simulink model "AE200_Landing_Gear_Model"  (R2021b)
settings: Solver=VariableStepAuto  StartTime=0.0  StopTime=10.0  RelTol=1e-3
settings Model: Creator=amazgrace  LastModifiedBy=amazgrace

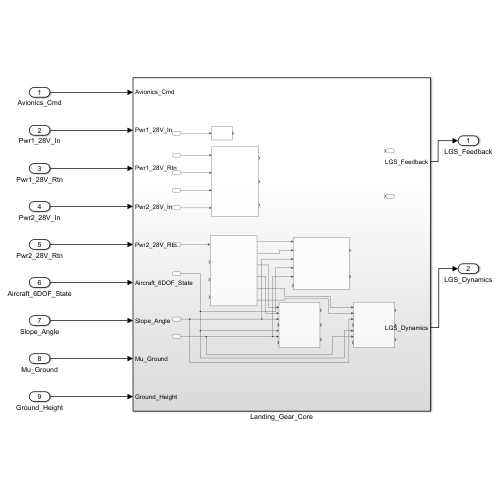
[thumbnail: Simulink's stored preview of the top-level diagram]
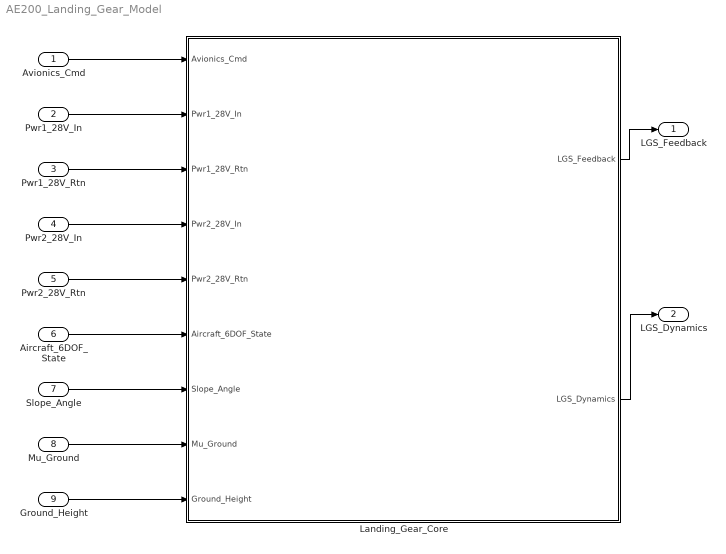
== system AE200_Landing_Gear_Model ==
  Avionics_Cmd : Inport
  Pwr1_28V_In : Inport  Port=2
  Pwr1_28V_Rtn : Inport  Port=3
  Pwr2_28V_In : Inport  Port=4
  Pwr2_28V_Rtn : Inport  Port=5
  Aircraft_6DOF_State : Inport  Port=6
  Slope_Angle : Inport  Port=7
  Mu_Ground : Inport  Port=8
  Ground_Height : Inport  Port=9
  Landing_Gear_Core : Subsystem
  LGS_Feedback : Outport
  LGS_Dynamics : Outport  Port=2
  wires:
  Avionics_Cmd/1 -> Landing_Gear_Core/1(Avionics_Cmd)
  Pwr1_28V_In/1 -> Landing_Gear_Core/2(Pwr1_28V_In)
  Pwr1_28V_Rtn/1 -> Landing_Gear_Core/3(Pwr1_28V_Rtn)
  Pwr2_28V_In/1 -> Landing_Gear_Core/4(Pwr2_28V_In)
  Pwr2_28V_Rtn/1 -> Landing_Gear_Core/5(Pwr2_28V_Rtn)
  Aircraft_6DOF_State/1 -> Landing_Gear_Core/6(Aircraft_6DOF_State)
  Landing_Gear_Core/2(LGS_Dynamics) -> LGS_Dynamics/1
  Landing_Gear_Core/1(LGS_Feedback) -> LGS_Feedback/1
  Slope_Angle/1 -> Landing_Gear_Core/7(Slope_Angle)
  Mu_Ground/1 -> Landing_Gear_Core/8(Mu_Ground)
  Ground_Height/1 -> Landing_Gear_Core/9(Ground_Height)

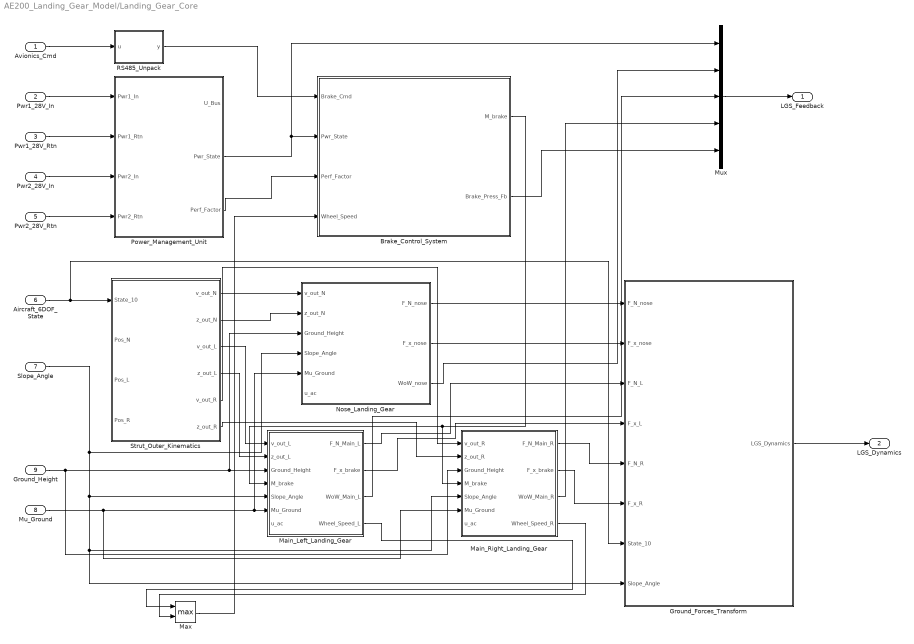
== system AE200_Landing_Gear_Model/Landing_Gear_Core ==
  Avionics_Cmd : Inport
  Pwr1_28V_In : Inport  Port=2
  Pwr1_28V_Rtn : Inport  Port=3
  Pwr2_28V_In : Inport  Port=4
  Pwr2_28V_Rtn : Inport  Port=5
  Aircraft_6DOF_State : Inport  Port=6
  Slope_Angle : Inport  Port=7
  Mu_Ground : Inport  Port=8
  Ground_Height : Inport  Port=9
  Brake_Control_System : Subsystem
  Ground_Forces_Transform : MATLAB Function  TreatAsAtomicUnit=on
  Main_Left_Landing_Gear : Subsystem
  Main_Right_Landing_Gear : Subsystem
  Max : MinMax  Function=max  Inputs=2
  Mux : Mux  Inputs=5
  Nose_Landing_Gear : Subsystem
  Power_Management_Unit : MATLAB Function  TreatAsAtomicUnit=on
  RS485_Unpack : MATLAB Function  TreatAsAtomicUnit=on
  Strut_Outer_Kinematics : MATLAB Function  TreatAsAtomicUnit=on
  LGS_Feedback : Outport
  LGS_Dynamics : Outport  Port=2
  wires:
  Avionics_Cmd/1 -> RS485_Unpack/1(u)
  Pwr1_28V_In/1 -> Power_Management_Unit/1(Pwr1_In)
  Pwr1_28V_Rtn/1 -> Power_Management_Unit/2(Pwr1_Rtn)
  Pwr2_28V_In/1 -> Power_Management_Unit/3(Pwr2_In)
  Pwr2_28V_Rtn/1 -> Power_Management_Unit/4(Pwr2_Rtn)
  Aircraft_6DOF_State/1 -> Ground_Forces_Transform/7(State_10), Strut_Outer_Kinematics/1(State_10)
  Strut_Outer_Kinematics/1(v_out_N) -> Nose_Landing_Gear/1(v_out_N)
  Strut_Outer_Kinematics/2(z_out_N) -> Nose_Landing_Gear/2(z_out_N)
  Strut_Outer_Kinematics/3(v_out_L) -> Main_Left_Landing_Gear/1(v_out_L)
  Strut_Outer_Kinematics/4(z_out_L) -> Main_Left_Landing_Gear/2(z_out_L)
  Slope_Angle/1 -> Ground_Forces_Transform/8(Slope_Angle), Main_Right_Landing_Gear/5(Slope_Angle), Main_Left_Landing_Gear/5(Slope_Angle), Nose_Landing_Gear/4(Slope_Angle)
  Strut_Outer_Kinematics/5(v_out_R) -> Main_Right_Landing_Gear/1(v_out_R)
  Strut_Outer_Kinematics/6(z_out_R) -> Main_Right_Landing_Gear/2(z_out_R)
  Mu_Ground/1 -> Nose_Landing_Gear/5(Mu_Ground), Main_Left_Landing_Gear/6(Mu_Ground), Main_Right_Landing_Gear/6(Mu_Ground)
  Ground_Height/1 -> Main_Right_Landing_Gear/3(Ground_Height), Nose_Landing_Gear/3(Ground_Height), Main_Left_Landing_Gear/3(Ground_Height)
  Nose_Landing_Gear/1(F_N_nose) -> Ground_Forces_Transform/1(F_N_nose)
  Nose_Landing_Gear/2(F_x_nose) -> Ground_Forces_Transform/2(F_x_nose)
  Main_Left_Landing_Gear/1(F_N_Main_L) -> Ground_Forces_Transform/3(F_N_L)
  Main_Left_Landing_Gear/2(F_x_brake) -> Ground_Forces_Transform/4(F_x_L)
  Main_Right_Landing_Gear/1(F_N_Main_R) -> Ground_Forces_Transform/5(F_N_R)
  Main_Right_Landing_Gear/2(F_x_brake) -> Ground_Forces_Transform/6(F_x_R)
  Ground_Forces_Transform/1(LGS_Dynamics) -> LGS_Dynamics/1
  Mux/1 -> LGS_Feedback/1
  Power_Management_Unit/2(Pwr_State) -> Brake_Control_System/2(Pwr_State), Mux/1
  Nose_Landing_Gear/3(WoW_nose) -> Mux/2
  Main_Left_Landing_Gear/3(WoW_Main_L) -> Mux/3
  Main_Right_Landing_Gear/3(WoW_Main_R) -> Mux/4
  RS485_Unpack/1(y) -> Brake_Control_System/1(Brake_Cmd)
  Power_Management_Unit/3(Perf_Factor) -> Brake_Control_System/3(Perf_Factor)
  Brake_Control_System/1(M_brake) -> Main_Right_Landing_Gear/4(M_brake), Main_Left_Landing_Gear/4(M_brake)
  Brake_Control_System/2(Brake_Press_Fb) -> Mux/5
  Main_Left_Landing_Gear/4(Wheel_Speed_L) -> Max/1
  Main_Right_Landing_Gear/4(Wheel_Speed_R) -> Max/2
  Max/1 -> Brake_Control_System/4(Wheel_Speed)

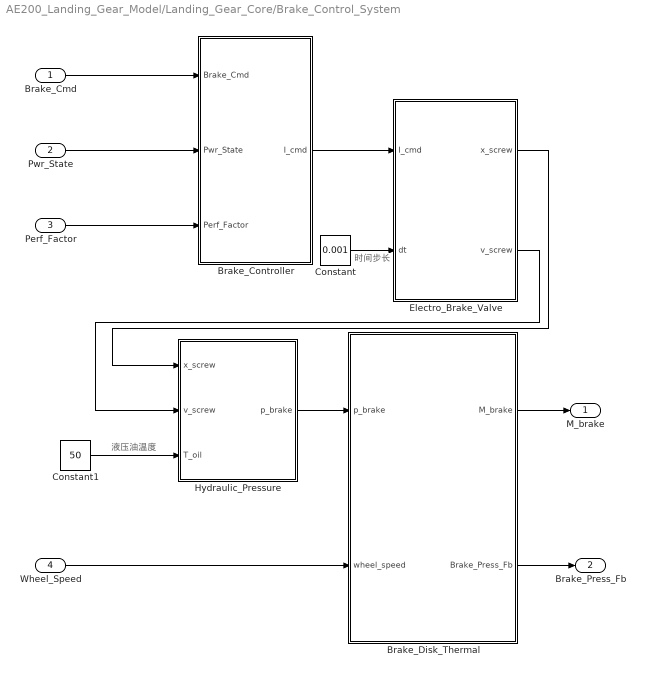
== system AE200_Landing_Gear_Model/Landing_Gear_Core/Brake_Control_System ==
  note: 时间步长
  note: 液压油温度
  Brake_Cmd : Inport
  Pwr_State : Inport  Port=2
  Perf_Factor : Inport  Port=3
  Wheel_Speed : Inport  Port=4
  Brake_Controller : MATLAB Function  TreatAsAtomicUnit=on
  Brake_Disk_Thermal : MATLAB Function  TreatAsAtomicUnit=on
  Constant : Constant  Value=0.001
  Constant1 : Constant  Value=50
  Electro_Brake_Valve : MATLAB Function  TreatAsAtomicUnit=on
  Hydraulic_Pressure : MATLAB Function  TreatAsAtomicUnit=on
  M_brake : Outport
  Brake_Press_Fb : Outport  Port=2
  wires:
  Brake_Cmd/1 -> Brake_Controller/1(Brake_Cmd)
  Pwr_State/1 -> Brake_Controller/2(Pwr_State)
  Perf_Factor/1 -> Brake_Controller/3(Perf_Factor)
  Brake_Controller/1(I_cmd) -> Electro_Brake_Valve/1(I_cmd)
  Brake_Disk_Thermal/2(Brake_Press_Fb) -> Brake_Press_Fb/1
  Brake_Disk_Thermal/1(M_brake) -> M_brake/1
  Electro_Brake_Valve/2(v_screw) -> Hydraulic_Pressure/2(v_screw)
  Hydraulic_Pressure/1(p_brake) -> Brake_Disk_Thermal/1(p_brake)
  Constant/1 -> Electro_Brake_Valve/2(dt)
  Constant1/1 -> Hydraulic_Pressure/3(T_oil)
  Wheel_Speed/1 -> Brake_Disk_Thermal/2(wheel_speed)
  Electro_Brake_Valve/1(x_screw) -> Hydraulic_Pressure/1(x_screw)

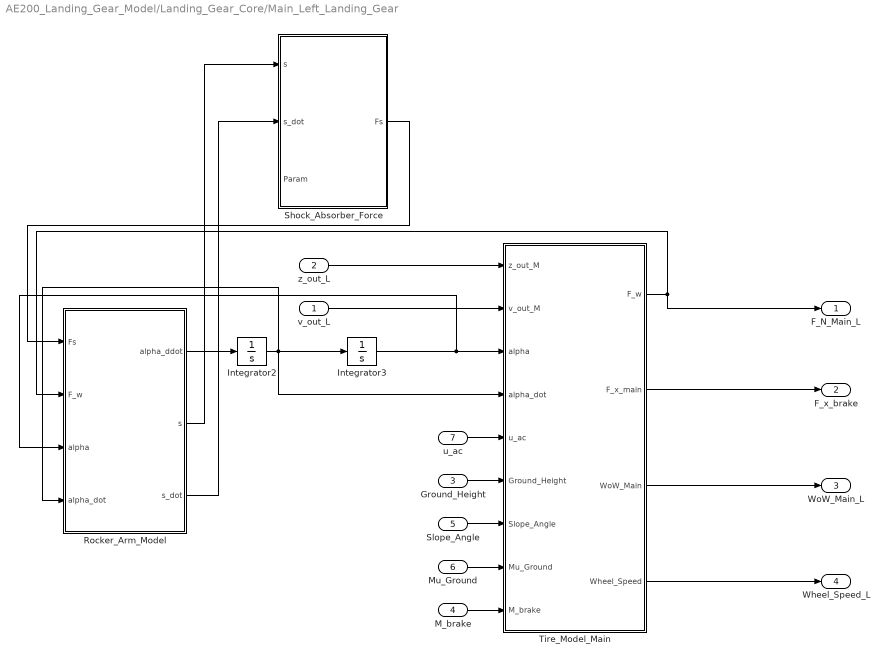
== system AE200_Landing_Gear_Model/Landing_Gear_Core/Main_Left_Landing_Gear ==
  v_out_L : Inport
  z_out_L : Inport  Port=2
  Ground_Height : Inport  Port=3
  M_brake : Inport  Port=4
  Slope_Angle : Inport  Port=5
  Mu_Ground : Inport  Port=6
  u_ac : Inport  Port=7
  Integrator2 : Integrator
  Integrator3 : Integrator
  Rocker_Arm_Model : MATLAB Function  TreatAsAtomicUnit=on
  Shock_Absorber_Force : MATLAB Function  TreatAsAtomicUnit=on
  Tire_Model_Main : MATLAB Function  TreatAsAtomicUnit=on
  F_N_Main_L : Outport
  F_x_brake : Outport  Port=2
  WoW_Main_L : Outport  Port=3
  Wheel_Speed_L : Outport  Port=4
  wires:
  v_out_L/1 -> Tire_Model_Main/2(v_out_M)
  Shock_Absorber_Force/1(Fs) -> Rocker_Arm_Model/1(Fs)
  Tire_Model_Main/1(F_w) -> F_N_Main_L/1, Rocker_Arm_Model/2(F_w)
  Rocker_Arm_Model/1(alpha_ddot) -> Integrator2/1
  Integrator2/1 -> Integrator3/1, Tire_Model_Main/4(alpha_dot), Rocker_Arm_Model/4(alpha_dot)
  Integrator3/1 -> Rocker_Arm_Model/3(alpha), Tire_Model_Main/3(alpha)
  z_out_L/1 -> Tire_Model_Main/1(z_out_M)
  Ground_Height/1 -> Tire_Model_Main/6(Ground_Height)
  Slope_Angle/1 -> Tire_Model_Main/7(Slope_Angle)
  Mu_Ground/1 -> Tire_Model_Main/8(Mu_Ground)
  M_brake/1 -> Tire_Model_Main/9(M_brake)
  u_ac/1 -> Tire_Model_Main/5(u_ac)
  Tire_Model_Main/3(WoW_Main) -> WoW_Main_L/1
  Rocker_Arm_Model/2(s) -> Shock_Absorber_Force/1(s)
  Rocker_Arm_Model/3(s_dot) -> Shock_Absorber_Force/2(s_dot)
  Tire_Model_Main/2(F_x_main) -> F_x_brake/1
  Tire_Model_Main/4(Wheel_Speed) -> Wheel_Speed_L/1

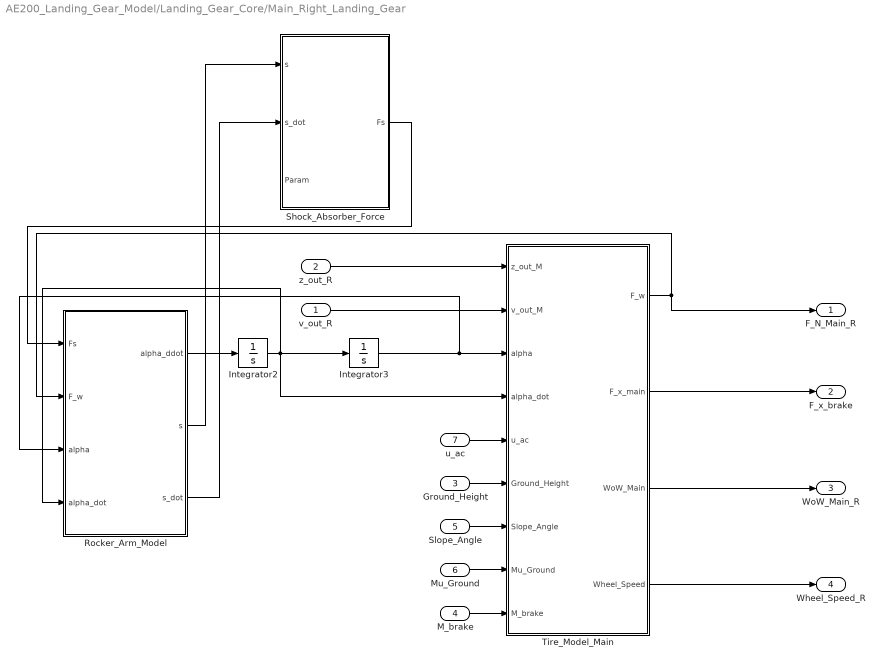
== system AE200_Landing_Gear_Model/Landing_Gear_Core/Main_Right_Landing_Gear ==
  v_out_R : Inport
  z_out_R : Inport  Port=2
  Ground_Height : Inport  Port=3
  M_brake : Inport  Port=4
  Slope_Angle : Inport  Port=5
  Mu_Ground : Inport  Port=6
  u_ac : Inport  Port=7
  Integrator2 : Integrator
  Integrator3 : Integrator
  Rocker_Arm_Model : MATLAB Function  TreatAsAtomicUnit=on
  Shock_Absorber_Force : MATLAB Function  TreatAsAtomicUnit=on
  Tire_Model_Main : MATLAB Function  TreatAsAtomicUnit=on
  F_N_Main_R : Outport
  F_x_brake : Outport  Port=2
  WoW_Main_R : Outport  Port=3
  Wheel_Speed_R : Outport  Port=4
  wires:
  Tire_Model_Main/3(WoW_Main) -> WoW_Main_R/1
  Integrator3/1 -> Rocker_Arm_Model/3(alpha), Tire_Model_Main/3(alpha)
  Mu_Ground/1 -> Tire_Model_Main/8(Mu_Ground)
  M_brake/1 -> Tire_Model_Main/9(M_brake)
  Integrator2/1 -> Integrator3/1, Tire_Model_Main/4(alpha_dot), Rocker_Arm_Model/4(alpha_dot)
  Tire_Model_Main/2(F_x_main) -> F_x_brake/1
  u_ac/1 -> Tire_Model_Main/5(u_ac)
  Rocker_Arm_Model/2(s) -> Shock_Absorber_Force/1(s)
  Rocker_Arm_Model/1(alpha_ddot) -> Integrator2/1
  Tire_Model_Main/1(F_w) -> F_N_Main_R/1, Rocker_Arm_Model/2(F_w)
  Ground_Height/1 -> Tire_Model_Main/6(Ground_Height)
  Rocker_Arm_Model/3(s_dot) -> Shock_Absorber_Force/2(s_dot)
  Shock_Absorber_Force/1(Fs) -> Rocker_Arm_Model/1(Fs)
  Slope_Angle/1 -> Tire_Model_Main/7(Slope_Angle)
  v_out_R/1 -> Tire_Model_Main/2(v_out_M)
  z_out_R/1 -> Tire_Model_Main/1(z_out_M)
  Tire_Model_Main/4(Wheel_Speed) -> Wheel_Speed_R/1

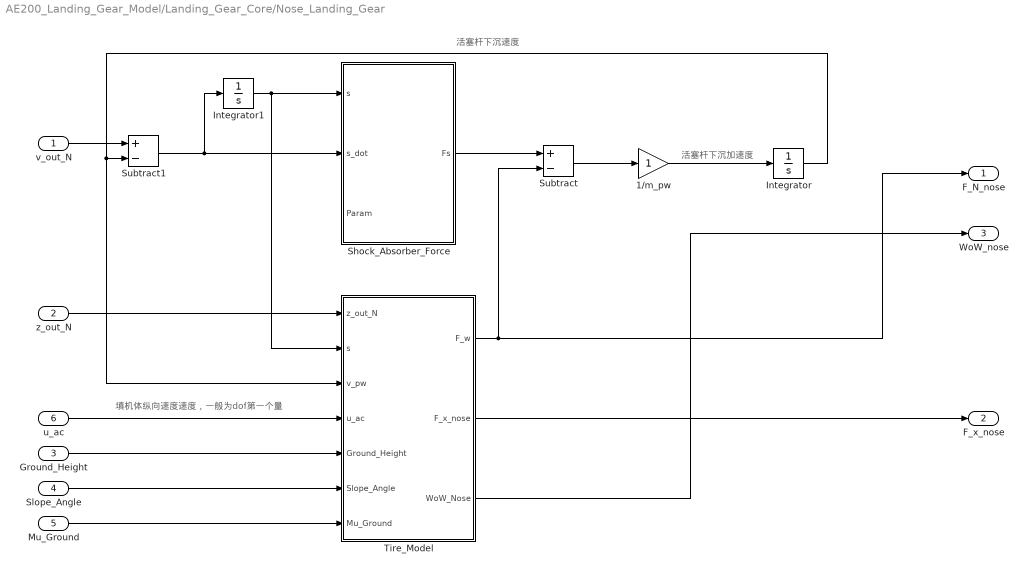
== system AE200_Landing_Gear_Model/Landing_Gear_Core/Nose_Landing_Gear ==
  note: 填机体纵向速度速度，一般为dof第一个量
  note: 活塞杆下沉加速度
  note: 活塞杆下沉速度
  v_out_N : Inport
  z_out_N : Inport  Port=2
  Ground_Height : Inport  Port=3
  Slope_Angle : Inport  Port=4
  Mu_Ground : Inport  Port=5
  u_ac : Inport  Port=6
  1/m_pw : Gain
  Integrator : Integrator
  Integrator1 : Integrator
  Shock_Absorber_Force : MATLAB Function  TreatAsAtomicUnit=on
  Subtract : Sum  Inputs=+-
  Subtract1 : Sum  Inputs=+-
  Tire_Model : MATLAB Function  TreatAsAtomicUnit=on
  F_N_nose : Outport
  F_x_nose : Outport  Port=2
  WoW_nose : Outport  Port=3
  wires:
  Shock_Absorber_Force/1(Fs) -> Subtract/1
  Subtract/1 -> 1/m_pw/1
  1/m_pw/1 -> Integrator/1
  v_out_N/1 -> Subtract1/1
  Integrator/1 -> Subtract1/2, Tire_Model/3(v_pw)
  Subtract1/1 -> Integrator1/1, Shock_Absorber_Force/2(s_dot)
  Integrator1/1 -> Tire_Model/2(s), Shock_Absorber_Force/1(s)
  z_out_N/1 -> Tire_Model/1(z_out_N)
  Tire_Model/3(WoW_Nose) -> WoW_nose/1
  Tire_Model/1(F_w) -> Subtract/2, F_N_nose/1
  Ground_Height/1 -> Tire_Model/5(Ground_Height)
  Slope_Angle/1 -> Tire_Model/6(Slope_Angle)
  Mu_Ground/1 -> Tire_Model/7(Mu_Ground)
  u_ac/1 -> Tire_Model/4(u_ac)
  Tire_Model/2(F_x_nose) -> F_x_nose/1

== matlab function AE200_Landing_Gear_Model/Landing_Gear_Core/Main_Right_Landing_Gear/Rocker_Arm_Model ==
  data: Fs input; alpha_ddot output; F_w input; alpha input; alpha_dot input; s output; s_dot output
function [alpha_ddot, s, s_dot] = Rocker_Arm_Model(Fs, F_w, alpha, alpha_dot)
% 普适主起落架摇臂运动模型 (对应文档 2.2.1 节)
% Fs: 缓冲器轴向力 (N)
% F_w: 地面垂直支持力 (N)
% alpha: 摇臂向上摆动转角 (rad), alpha_dot: 摇臂角速度 (rad/s)

% --- 1. 摇臂几何与惯量参数（后续可按实际图纸修改） ---
L_w     = 0.45;   % 摇臂枢轴到主轮轮心的杆长 (m)
L_s     = 0.18;   % 摇臂枢轴到缓冲器下铰点的力臂长 (m)
alpha_0 = 0.35;   % 缓冲器未压缩时摇臂初始下偏角 (rad, 约20度)
J_arm   = 3.5;    % 摇臂与机轮绕枢轴的等效转动惯量 (kg*m^2)
C_pivot = 15.0;   % 摇臂转轴结构阻尼系数 (N*m*s/rad，增加数值稳定性)

% --- 2. 计算实时力臂与转动微分方程 ---
% 限制转角在合理物理范围 [-0.05, 0.8] rad 内计算三角函数
alpha_eff = min(max(-0.05, alpha), 0.8);

% 地面支持力产生的转动力矩 M_ground 与 缓冲器产生的阻力矩 M_strut
M_ground = F_w * L_w * cos(alpha_0 - alpha_eff);
M_strut  = Fs  * L_s * cos(alpha_eff);

% 求解摇臂角加速度 alpha_ddot
alpha_ddot = (M_ground - M_strut - C_pivot * alpha_dot) / J_arm;

% --- 3. 几何转换：由摇臂转角求缓冲器压缩量 s 与压缩速度 s_dot ---
s     = L_s * sin(alpha_eff);
s_dot = L_s * cos(alpha_eff) * alpha_dot;
end

== matlab function AE200_Landing_Gear_Model/Landing_Gear_Core/Main_Right_Landing_Gear/Shock_Absorber_Force ==
  data: s input; Fs output; s_dot input; Param input
function Fs = Shock_Absorber_Force(s, s_dot, Param)
% 输入：s (压缩量, m), s_dot (压缩速度, m/s)
% Param 结构体包含: Aa, P0, V0, n, Patm, rho_oil, Ao, Ad, Cd, k_st, s_max

% 1. 空气弹簧力 Fair (限制 s_eff 在 [0, 0.99*V0/Aa] 之间防止分母为0或负压异常)
s_eff = min(max(0, s), 0.99 * Param.V0 / Param.Aa);
Fair = Param.Aa * (Param.P0 * (Param.V0 / (Param.V0 - Param.Aa * s_eff))^Param.n - Param.Patm);
Fair = max(0, Fair); % 保证弹簧力非负

% 2. 油液阻尼力 Foil
K_oil = (Param.rho_oil * Param.Ao^3) / (2 * Param.Cd^2 * Param.Ad^2);
Foil = s_dot * abs(s_dot) * K_oil;

% 3. 内部摩擦力 Ff
Ff = 0.06 * Fair * sign(s_dot);

% 4. 结构限制力 Fst
if s < 0
    Fst = Param.k_st * s;
elseif s <= Param.s_max
    Fst = 0;
else
    Fst = Param.k_st * (s - Param.s_max);
end

% 5. 缓冲器内部合力 Fs
Fs = Fair + Foil + Ff + Fst;
end

== matlab function AE200_Landing_Gear_Model/Landing_Gear_Core/Main_Right_Landing_Gear/Tire_Model_Main ==
  data: z_out_M input; F_w output; v_out_M input; alpha input; alpha_dot input; u_ac input; Ground_Height input; Slope_Angle input; Mu_Ground input; M_brake input; F_x_main output; WoW_Main output; Wheel_Speed output
function [F_w, F_x_main, WoW_Main, Wheel_Speed] = Tire_Model_Main(z_out_M, v_out_M, alpha, alpha_dot, u_ac, Ground_Height, Slope_Angle, Mu_Ground, M_brake)
% 普适主起落架轮胎模型（含高度、坡度、地面静摩擦系数与静刹车力矩耦合）

% --- 1. 主轮与安装参数 ---
L_m0    = 1.05;   % 外筒基准点到摇臂枢轴的垂直距离 (m)
L_w     = 0.45;   % 摇臂杆长 (m)
alpha_0 = 0.35;   % 摇臂初始角 (rad)
R_tire0 = 0.30;   % 主轮自由半径 (m)
K_t     = 6e5;    % 主轮轮胎径向刚度 (N/m)
C_t     = 3000;   % 主轮轮胎径向阻尼 (N*s/m)
WoW_Thr = 500;    % 主轮载开关触发阈值 (N)
x_main  = -0.8;   % 主起落架相对于飞机重心的纵向安装坐标 x (m，重心后方为负)
mu_roll = 0.015;  % 无刹车时的滚动摩擦系数

% --- 2. 计算主轮触地点处的实际地面高度 Ground_z（含高度与坡度） ---
Ground_z = Ground_Height - x_main * tan(Slope_Angle);

% --- 3. 由摇臂转角 alpha 计算主轮最低点高度与下沉速度 ---
alpha_eff = min(max(-0.05, alpha), 0.8);
% 轮心高度 = 外筒高度 + 枢轴距离 + 摇臂垂向投影 + 轮胎半径
z_tire_bottom = z_out_M + L_m0 + L_w * sin(alpha_0 - alpha_eff) + R_tire0;
% 轮心下沉速度 = 外筒下沉速度 - 摇臂上摆引起的轮心上升速度
v_wheel_down  = v_out_M - L_w * cos(alpha_0 - alpha_eff) * alpha_dot;

% --- 4. 计算轮胎法向压缩量 delta_t 与垂直支持力 F_w ---
delta_t = (z_tire_bottom - Ground_z) * cos(Slope_Angle);

if delta_t > 0
    delta_t_dot = v_wheel_down * cos(Slope_Angle);
    F_w = max(0, K_t * delta_t + C_t * delta_t_dot);
else
    delta_t = 0;
    F_w = 0;
end

% --- 5. 计算静刹车力矩与地面静摩擦系数耦合的纵向力 F_x_main ---
if F_w > 0
    % 轮胎受压后的有效滚动半径 (防过压保护下限 0.1m)
    R_eff = max(0.1, R_tire0 - 0.33 * delta_t);
    
    % (A) 地面静摩擦系数决定的最大静摩擦力上限
    F_ground_limit = max(0, Mu_Ground) * F_w;
    
    % (B) 刹车力矩决定的制动力上限 + 基础滚动摩阻
    F_brake_limit  = max(0, M_brake) / R_eff + mu_roll * F_w;
    
    % 实际能提供的最大驻停静摩擦力取 (A) 和 (B) 的较小值
    F_hold_max = min(F_ground_limit, F_brake_limit);
    
    % 考虑坡道重力下滑趋势与飞机微动速度 u_ac 合成滑移趋势
    % 当飞机在坡道停放或有微动速度时，输出反向静摩擦力抵抗运动
    u_trend = u_ac - 0.02 * sin(Slope_Angle); 
    F_x_main = - F_hold_max * tanh(u_trend / 0.005);
else
    F_x_main = 0;
end

% --- 6. 主轮载开关判定 ---
WoW_Main = (F_w >= WoW_Thr);

% --- 7. 计算主轮轮速 wheel_speed (rad/s) ---
if F_w > 0
    R_eff = max(0.1, R_tire0 - 0.33 * delta_t);
    % 若刹车力矩大于地面摩擦力矩上限（车轮抱死驻停），则轮速为 0；否则为滚动角速度
    if M_brake >= F_ground_limit * R_eff
        Wheel_Speed = 0; % 驻停刹死状态，车轮不转
    else
        Wheel_Speed = abs(u_ac) / R_eff;
    end
else
    Wheel_Speed = 0; % 空中悬空状态，轮速为 0
end

end

== matlab function AE200_Landing_Gear_Model/Landing_Gear_Core/Ground_Forces_Transform ==
  data: F_N_nose input; LGS_Dynamics output; F_x_nose input; F_N_L input; F_x_L input; F_N_R input; F_x_R input; State_10 input; Slope_Angle input
function LGS_Dynamics = Ground_Forces_Transform(F_N_nose, F_x_nose, F_N_L, F_x_L, F_N_R, F_x_R, State_10, Slope_Angle)
% 汇总前、左主、右主起落架地面作用力与力矩，并通过 Lbw 转换至飞机机体坐标系
% 输出 LGS_Dynamics: [6x1] 向量 [Fx_b; Fy_b; Fz_b; Mx_b; My_b; Mz_b]

% --- 1. 提取飞机姿态角 (NED坐标系) ---
phi   = State_10(7); % 滚转角 (rad)
theta = State_10(8); % 俯仰角 (rad)

% --- 2. 起落架触地点相对于飞机重心的力臂坐标 [x, y, z] (m) ---
r_N = [ 2.5,  0.0, 1.5]; % 前轮触地点近似力臂
r_L = [-0.8, -1.2, 1.5]; % 左主轮触地点近似力臂
r_R = [-0.8,  1.2, 1.5]; % 右主轮触地点近似力臂

% --- 3. 在坡面/地面坐标系下合成三轴地面力 (NED：X向前，Y向右，Z向下) ---
% 注意：支持力 F_N 方向垂直地面向上，因此在向下为正的 Z 轴中取负号！
Fw_N = [F_x_nose; 0; -F_N_nose];
Fw_L = [F_x_L;    0; -F_N_L];
Fw_R = [F_x_R;    0; -F_N_R];

% 地面系总合力 F_ground (3x1)
F_ground = Fw_N + Fw_L + Fw_R;

% --- 4. 坐标转换矩阵 L_bw：将地面/坡面系作用力转换到飞机机体坐标系 ---
% 有效俯仰角（叠加地面坡度角 Slope_Angle）
theta_eff = theta - Slope_Angle;

L_bw = [ cos(theta_eff),                  0,                 -sin(theta_eff);
         sin(phi)*sin(theta_eff),  cos(phi),  sin(phi)*cos(theta_eff);
         cos(phi)*sin(theta_eff), -sin(phi),  cos(phi)*cos(theta_eff) ];

% 转换各轮地面力到机体坐标系
Fb_N = L_bw * Fw_N;
Fb_L = L_bw * Fw_L;
Fb_R = L_bw * Fw_R;

% 机体坐标系下的三轴总地面作用力 [Fx_b; Fy_b; Fz_b]
F_body = Fb_N + Fb_L + Fb_R;

% --- 5. 计算地面作用力对飞机重心的三轴力矩 M = r x F [Mx_b; My_b; Mz_b] ---
M_body = cross(r_N', Fb_N) + cross(r_L', Fb_L) + cross(r_R', Fb_R);

% --- 6. 组合为 6 维动力学向量输出给 6DOF ---
LGS_Dynamics = [F_body; M_body];
end

== matlab function AE200_Landing_Gear_Model/Landing_Gear_Core/Brake_Control_System/Brake_Controller ==
  data: Brake_Cmd input; I_cmd output; Pwr_State input; Perf_Factor input
function I_cmd = Brake_Controller(Brake_Cmd, Pwr_State, Perf_Factor)
% 刹车控制器逻辑
if Pwr_State == 0
    I_cmd = 0.0; % 掉电失效，电流归零
else
    % 正常或降级工况：根据指令计算理论控制电流，并受供电性能系数折减
    I_nominal = Brake_Cmd * 1.5; % 假设满指令对应 1.5A 额定控制电流
    I_cmd = I_nominal * Perf_Factor;
end
end

== matlab function AE200_Landing_Gear_Model/Landing_Gear_Core/Brake_Control_System/Electro_Brake_Valve ==
  data: I_cmd input; x_screw output; dt input; v_screw output
function [x_screw, v_screw] = Electro_Brake_Valve(I_cmd, dt)
% 滚珠丝杠作动模型简化实现 (使用 persistent 状态记忆位移)
persistent x v;
if isempty(x), x = 0; v = 0; end

% 简单的惯性环节跟随电流指令
v_target = I_cmd * 0.02; % 比例系数
v = v + (v_target - v) * 0.2; 
x = x + v * 0.1;
x_screw = max(0, x); % 丝杠位移限制非负
v_screw = v;
end

== matlab function AE200_Landing_Gear_Model/Landing_Gear_Core/Power_Management_Unit ==
  data: Pwr1_In input; U_Bus output; Pwr1_Rtn input; Pwr2_In input; Pwr2_Rtn input; Pwr_State output; Perf_Factor output
function [U_Bus, Pwr_State, Perf_Factor] = Power_Monitor(Pwr1_In, Pwr1_Rtn, Pwr2_In, Pwr2_Rtn)
% ATS-GDS-06-001C 低压供电及用电特性模拟模块

% 1. 回线（地线）有效性检查：正常回线电压应在 0V 附近（容差 ±2V）
% 若注入回线断开故障（如给 NaN 或 28V 浮空电平），则判定该通道无效
if isnan(Pwr1_Rtn) || abs(Pwr1_Rtn) > 2.0
    U1_eff = 0;
else
    U1_eff = max(0, Pwr1_In - Pwr1_Rtn);
end

if isnan(Pwr2_Rtn) || abs(Pwr2_Rtn) > 2.0
    U2_eff = 0;
else
    U2_eff = max(0, Pwr2_In - Pwr2_Rtn);
end

% 2. 双余度供电汇流（二极管“或”逻辑，取两路中较高的有效电压）
U_Bus = max(U1_eff, U2_eff);

% 3. 根据 ATS-GDS-06-001C 电压区间计算状态与性能降级系数
if U_Bus >= 22.0 && U_Bus <= 30.3
    % 【正常工作区】：22V ~ 30.3V
    Pwr_State = uint8(2);
    Perf_Factor = 1.0;
    
elseif U_Bus >= 18.0 && U_Bus < 22.0
    % 【性能降级区】：18V ~ 22V
    Pwr_State = uint8(1);
    % 方式A（推荐，物理意义明确）：按实际电压与额定最低正常电压(22V)之比进行折减
    % 18V 时约为 18/22 = 0.8182 (即最大控制电流/电磁力矩下降约18.2%)
    Perf_Factor = U_Bus / 22.0; 
    % 注：若要求在 18~22V 之间从 0.5 线性变化到 1.0，可改为：
    % Perf_Factor = 0.5 + 0.5 * (U_Bus - 18.0) / (22.0 - 18.0);
    
elseif U_Bus > 30.3 && U_Bus <= 32.0
    % 【过压容忍/轻微降级区】（可根据具体规范微调）
    Pwr_State = uint8(1);
    Perf_Factor = 1.0;
    
else
    % 【功能失效区】：低于 18V 欠压失效，或高于 32V 过压保护切断
    Pwr_State = uint8(0);
    Perf_Factor = 0.0;
end

== matlab function AE200_Landing_Gear_Model/Landing_Gear_Core/Brake_Control_System/Hydraulic_Pressure ==
  data: x_screw input; v_screw input; p_brake output; T_oil input
function p_brake = Hydraulic_Pressure(x_screw, v_screw, T_oil)
% 对应文档 2.4.4 液压力计算模块
persistent p T_prev;
if isempty(p)
    p = 0; 
    T_prev = T_oil;
end

dt = 0.001;          % 仿真步长 (s)
B  = 1.2e9;          % 液压油体积弹性模量 (Pa)
V  = 5.0e-4;         % 刹车油路总容积 (m^3)
alpha_oil = 0.0007;  % 液压油热膨胀系数 (1/℃)
A_screw   = 2.0e-4;  % 丝杠活塞等效截面积 (m^2)
K_leak    = 1.0e-13; % 驻停刹车内部微漏油系数 (m^3/(s*Pa)，模拟断电后静刹车力矩随时间缓慢衰减)
K_comp    = 1.5e-11; % 刹车装置轴向刚度与管路弹性柔度系数 (m^3/Pa)

% 1. 判断滚珠丝杠是否回退到初始位置（松刹车与油杯连通补油/泄压）
if x_screw <= 1e-5 && v_screw <= 0
    p = 0; % 与油杯连通，压差消除
else
    % 2. Q1: 液压油流入流出体积速率（考虑丝杠回退补油与高压漏油衰减）
    Q1 = - K_leak * p;

    % 3. Q2: 刹车油路容积变化速率（由丝杠运动速度 v_screw 决定，并考虑管路/卡钳弹性等效系数）
    Q2 = A_screw * v_screw;

    % 4. 温度变化速率 dT/dt
    dT_dt = (T_oil - T_prev) / dt;

    % 5. 文档公式：dp/dt = (B/V)*(Q1 + Q2) + alpha*B*(dT/dt)
    % 计入管路与刹车装置轴向弹性引起的容积变化修正分母 (1 + (B/V)*K_comp)
    dp_dt = ((B / V) * (Q1 + Q2) + alpha_oil * B * dT_dt) / (1 + (B / V) * K_comp);

    p = max(0, p + dp_dt * dt);
end

T_prev = T_oil;
p_brake = p / 1e6; % 转换为 MPa 输出
end

== matlab function AE200_Landing_Gear_Model/Landing_Gear_Core/Brake_Control_System/Brake_Disk_Thermal ==
  data: p_brake input; M_brake output; wheel_speed input; Brake_Press_Fb output
function [M_brake, Brake_Press_Fb] = Brake_Disk_Thermal(p_brake, wheel_speed)
% 刹车盘力矩与压力反馈计算

% 基础参数
A_piston = 0.02;   % 活塞有效面积 (m^2)
R_mean   = 0.15;   % 摩擦片平均摩擦半径 (m)
N_surfaces = 4;    % 摩擦面对数
mu_base  = 0.35;   % 基础摩擦系数

% 夹紧力 = 压力 * 活塞面积
F_clamp = p_brake * 1e6 * A_piston;

% 刹车力矩 = 夹紧力 * 摩擦半径 * 摩擦对数 * 摩擦系数
M_brake = F_clamp * R_mean * N_surfaces * mu_base;

% 压力反馈给控制器或顶层总线
Brake_Press_Fb = p_brake; 
end

== matlab function AE200_Landing_Gear_Model/Landing_Gear_Core/RS485_Unpack ==
  data: u input; y output
function y = fcn(u)

y = u;

== matlab function AE200_Landing_Gear_Model/Landing_Gear_Core/Strut_Outer_Kinematics ==
  data: State_10 input; v_out_N output; Pos_N input; Pos_L input; Pos_R input; z_out_N output; v_out_L output; z_out_L output; v_out_R output; z_out_R output
function [v_out_N, z_out_N, v_out_L, z_out_L, v_out_R, z_out_R] = Strut_Outer_Kinematics(State_10, Pos_N, Pos_L, Pos_R)
% State_10: [u, v, w, p, q, r, phi, theta, psi, Pz]
% Pos_N, Pos_L, Pos_R: 前、左、右起落架在机体系下的安装坐标 [x, y, z]

u = State_10(1); v = State_10(2); w = State_10(3);
p = State_10(4); q = State_10(5); r = State_10(6);
phi = State_10(7); theta = State_10(8); Pz = State_10(10);

% 辅助子函数计算单个起落架外筒状态
[v_out_N, z_out_N] = calc_single(u,v,w, p,q,r, phi,theta, Pz, Pos_N);
[v_out_L, z_out_L] = calc_single(u,v,w, p,q,r, phi,theta, Pz, Pos_L);
[v_out_R, z_out_R] = calc_single(u,v,w, p,q,r, phi,theta, Pz, Pos_R);
end

function [v_out, z_out] = calc_single(u,v,w, p,q,r, phi,theta, Pz, pos)
xg = pos(1); yg = pos(2); zg = pos(3);
ug = u + q*zg - r*yg;
vg = v + r*xg - p*zg;
wg = w + p*yg - q*xg;

v_out = -ug*sin(theta) + vg*sin(phi)*cos(theta) + wg*cos(phi)*cos(theta);
z_out = Pz - xg*sin(theta) + yg*sin(phi)*cos(theta) + zg*cos(phi)*cos(theta);
end

== matlab function AE200_Landing_Gear_Model/Landing_Gear_Core/Nose_Landing_Gear/Shock_Absorber_Force ==
  data: s input; Fs output; s_dot input; Param input
function Fs = Shock_Absorber_Force(s, s_dot, Param)
% 输入：s (压缩量, m), s_dot (压缩速度, m/s)
% Param 结构体包含: Aa, P0, V0, n, Patm, rho_oil, Ao, Ad, Cd, k_st, s_max

% 1. 空气弹簧力 Fair (限制 s_eff 在 [0, 0.99*V0/Aa] 之间防止分母为0或负压异常)
s_eff = min(max(0, s), 0.99 * Param.V0 / Param.Aa);
Fair = Param.Aa * (Param.P0 * (Param.V0 / (Param.V0 - Param.Aa * s_eff))^Param.n - Param.Patm);
Fair = max(0, Fair); % 保证弹簧力非负

% 2. 油液阻尼力 Foil
K_oil = (Param.rho_oil * Param.Ao^3) / (2 * Param.Cd^2 * Param.Ad^2);
Foil = s_dot * abs(s_dot) * K_oil;

% 3. 内部摩擦力 Ff
Ff = 0.06 * Fair * sign(s_dot);

% 4. 结构限制力 Fst
if s < 0
    Fst = Param.k_st * s;
elseif s <= Param.s_max
    Fst = 0;
else
    Fst = Param.k_st * (s - Param.s_max);
end

% 5. 缓冲器内部合力 Fs
Fs = Fair + Foil + Ff + Fst;
end

== matlab function AE200_Landing_Gear_Model/Landing_Gear_Core/Main_Left_Landing_Gear/Shock_Absorber_Force ==
  data: s input; Fs output; s_dot input; Param input
function Fs = Shock_Absorber_Force(s, s_dot, Param)
% 输入：s (压缩量, m), s_dot (压缩速度, m/s)
% Param 结构体包含: Aa, P0, V0, n, Patm, rho_oil, Ao, Ad, Cd, k_st, s_max

% 1. 空气弹簧力 Fair (限制 s_eff 在 [0, 0.99*V0/Aa] 之间防止分母为0或负压异常)
s_eff = min(max(0, s), 0.99 * Param.V0 / Param.Aa);
Fair = Param.Aa * (Param.P0 * (Param.V0 / (Param.V0 - Param.Aa * s_eff))^Param.n - Param.Patm);
Fair = max(0, Fair); % 保证弹簧力非负

% 2. 油液阻尼力 Foil
K_oil = (Param.rho_oil * Param.Ao^3) / (2 * Param.Cd^2 * Param.Ad^2);
Foil = s_dot * abs(s_dot) * K_oil;

% 3. 内部摩擦力 Ff
Ff = 0.06 * Fair * sign(s_dot);

% 4. 结构限制力 Fst
if s < 0
    Fst = Param.k_st * s;
elseif s <= Param.s_max
    Fst = 0;
else
    Fst = Param.k_st * (s - Param.s_max);
end

% 5. 缓冲器内部合力 Fs
Fs = Fair + Foil + Ff + Fst;
end

== matlab function AE200_Landing_Gear_Model/Landing_Gear_Core/Nose_Landing_Gear/Tire_Model ==
  data: z_out_N input; F_w output; F_x_nose output; s input; v_pw input; u_ac input; Ground_Height input; Slope_Angle input; WoW_Nose output; Mu_Ground input
function [F_w, F_x_nose, WoW_Nose] = Tire_Model_Nose(z_out_N, s, v_pw, u_ac, Ground_Height, Slope_Angle, Mu_Ground)
% 输入新增：
% u_ac: 飞机机体纵向速度 u (m/s)，来自6DOF状态第1个量
% Mu_Ground: 地面静摩擦/滑动摩擦系数 (如 0.1 ~ 0.8)
% 输出新增：
% F_x_nose: 前轮受到的地面纵向摩擦力 (N)

% --- 1. 轮胎与结构参数 ---
L_strut0 = 1.2;    % 未压缩时外筒到轮心距离 (m)
R_tire0  = 0.25;   % 前轮自由半径 (m)
K_t      = 4e5;    % 轮胎径向刚度 (N/m)
C_t      = 2000;   % 轮胎径向阻尼 (N*s/m)
WoW_Thr  = 200;    % 轮载开关阈值 (N)
x_nose   = 2.5;    % 前起纵向安装坐标 (m)
mu_roll  = 0.02;   % 前轮无刹车时的基准滚动摩阻系数

% --- 2. 计算实际地面高度与轮胎压缩量 ---
Ground_z = Ground_Height - x_nose * tan(Slope_Angle);
z_tire_bottom = z_out_N + (L_strut0 + R_tire0) - s;
delta_t = (z_tire_bottom - Ground_z) * cos(Slope_Angle);

% --- 3. 计算垂直支持力 F_w ---
if delta_t > 0
    delta_t_dot = v_pw * cos(Slope_Angle);
    F_w = max(0, K_t * delta_t + C_t * delta_t_dot);
else
    F_w = 0;
end

% --- 4. 计算考虑地面摩擦系数 Mu_Ground 的纵向摩擦力 F_x_nose ---
if F_w > 0
    % 地面能提供的最大静摩擦力上限 = 地面摩擦系数 * 垂直支持力
    F_friction_max = Mu_Ground * F_w;
    
    % 前轮无刹车装置，纵向阻力由滚动摩阻提供，但绝不能超过地面最大摩擦上限
    % (例如在极滑冰面 Mu_Ground < 0.02 时，受 Mu_Ground 限制)
    mu_eff = min(mu_roll, Mu_Ground);
    
    % 使用平滑 tanh 函数替代 sign(u_ac)，防止静止 (u_ac=0) 时在 Simulink 中产生高频抖振
    F_x_nose = - mu_eff * F_w * tanh(u_ac / 0.01);
else
    F_x_nose = 0;
end

% --- 5. 轮载开关判断 ---
WoW_Nose = (F_w >= WoW_Thr);
end

== matlab function AE200_Landing_Gear_Model/Landing_Gear_Core/Main_Left_Landing_Gear/Rocker_Arm_Model ==
  data: Fs input; alpha_ddot output; F_w input; alpha input; alpha_dot input; s output; s_dot output
function [alpha_ddot, s, s_dot] = Rocker_Arm_Model(Fs, F_w, alpha, alpha_dot)
% 普适主起落架摇臂运动模型 (对应文档 2.2.1 节)
% Fs: 缓冲器轴向力 (N)
% F_w: 地面垂直支持力 (N)
% alpha: 摇臂向上摆动转角 (rad), alpha_dot: 摇臂角速度 (rad/s)

% --- 1. 摇臂几何与惯量参数（后续可按实际图纸修改） ---
L_w     = 0.45;   % 摇臂枢轴到主轮轮心的杆长 (m)
L_s     = 0.18;   % 摇臂枢轴到缓冲器下铰点的力臂长 (m)
alpha_0 = 0.35;   % 缓冲器未压缩时摇臂初始下偏角 (rad, 约20度)
J_arm   = 3.5;    % 摇臂与机轮绕枢轴的等效转动惯量 (kg*m^2)
C_pivot = 15.0;   % 摇臂转轴结构阻尼系数 (N*m*s/rad，增加数值稳定性)

% --- 2. 计算实时力臂与转动微分方程 ---
% 限制转角在合理物理范围 [-0.05, 0.8] rad 内计算三角函数
alpha_eff = min(max(-0.05, alpha), 0.8);

% 地面支持力产生的转动力矩 M_ground 与 缓冲器产生的阻力矩 M_strut
M_ground = F_w * L_w * cos(alpha_0 - alpha_eff);
M_strut  = Fs  * L_s * cos(alpha_eff);

% 求解摇臂角加速度 alpha_ddot
alpha_ddot = (M_ground - M_strut - C_pivot * alpha_dot) / J_arm;

% --- 3. 几何转换：由摇臂转角求缓冲器压缩量 s 与压缩速度 s_dot ---
s     = L_s * sin(alpha_eff);
s_dot = L_s * cos(alpha_eff) * alpha_dot;
end

== matlab function AE200_Landing_Gear_Model/Landing_Gear_Core/Main_Left_Landing_Gear/Tire_Model_Main ==
  data: z_out_M input; F_w output; v_out_M input; alpha input; alpha_dot input; u_ac input; Ground_Height input; Slope_Angle input; Mu_Ground input; M_brake input; F_x_main output; WoW_Main output; Wheel_Speed output
function [F_w, F_x_main, WoW_Main, Wheel_Speed] = Tire_Model_Main(z_out_M, v_out_M, alpha, alpha_dot, u_ac, Ground_Height, Slope_Angle, Mu_Ground, M_brake)
% 普适主起落架轮胎模型（含高度、坡度、地面静摩擦系数与静刹车力矩耦合）

% --- 1. 主轮与安装参数 ---
L_m0    = 1.05;   % 外筒基准点到摇臂枢轴的垂直距离 (m)
L_w     = 0.45;   % 摇臂杆长 (m)
alpha_0 = 0.35;   % 摇臂初始角 (rad)
R_tire0 = 0.30;   % 主轮自由半径 (m)
K_t     = 6e5;    % 主轮轮胎径向刚度 (N/m)
C_t     = 3000;   % 主轮轮胎径向阻尼 (N*s/m)
WoW_Thr = 500;    % 主轮载开关触发阈值 (N)
x_main  = -0.8;   % 主起落架相对于飞机重心的纵向安装坐标 x (m，重心后方为负)
mu_roll = 0.015;  % 无刹车时的滚动摩擦系数

% --- 2. 计算主轮触地点处的实际地面高度 Ground_z（含高度与坡度） ---
Ground_z = Ground_Height - x_main * tan(Slope_Angle);

% --- 3. 由摇臂转角 alpha 计算主轮最低点高度与下沉速度 ---
alpha_eff = min(max(-0.05, alpha), 0.8);
% 轮心高度 = 外筒高度 + 枢轴距离 + 摇臂垂向投影 + 轮胎半径
z_tire_bottom = z_out_M + L_m0 + L_w * sin(alpha_0 - alpha_eff) + R_tire0;
% 轮心下沉速度 = 外筒下沉速度 - 摇臂上摆引起的轮心上升速度
v_wheel_down  = v_out_M - L_w * cos(alpha_0 - alpha_eff) * alpha_dot;

% --- 4. 计算轮胎法向压缩量 delta_t 与垂直支持力 F_w ---
delta_t = (z_tire_bottom - Ground_z) * cos(Slope_Angle);

if delta_t > 0
    delta_t_dot = v_wheel_down * cos(Slope_Angle);
    F_w = max(0, K_t * delta_t + C_t * delta_t_dot);
else
    delta_t = 0;
    F_w = 0;
end

% --- 5. 计算静刹车力矩与地面静摩擦系数耦合的纵向力 F_x_main ---
if F_w > 0
    % 轮胎受压后的有效滚动半径 (防过压保护下限 0.1m)
    R_eff = max(0.1, R_tire0 - 0.33 * delta_t);
    
    % (A) 地面静摩擦系数决定的最大静摩擦力上限
    F_ground_limit = max(0, Mu_Ground) * F_w;
    
    % (B) 刹车力矩决定的制动力上限 + 基础滚动摩阻
    F_brake_limit  = max(0, M_brake) / R_eff + mu_roll * F_w;
    
    % 实际能提供的最大驻停静摩擦力取 (A) 和 (B) 的较小值
    F_hold_max = min(F_ground_limit, F_brake_limit);
    
    % 考虑坡道重力下滑趋势与飞机微动速度 u_ac 合成滑移趋势
    % 当飞机在坡道停放或有微动速度时，输出反向静摩擦力抵抗运动
    u_trend = u_ac - 0.02 * sin(Slope_Angle); 
    F_x_main = - F_hold_max * tanh(u_trend / 0.005);
else
    F_x_main = 0;
end

% --- 6. 主轮载开关判定 ---
WoW_Main = (F_w >= WoW_Thr);

% --- 7. 计算主轮轮速 wheel_speed (rad/s) ---
if F_w > 0
    R_eff = max(0.1, R_tire0 - 0.33 * delta_t);
    % 若刹车力矩大于地面摩擦力矩上限（车轮抱死驻停），则轮速为 0；否则为滚动角速度
    if M_brake >= F_ground_limit * R_eff
        Wheel_Speed = 0; % 驻停刹死状态，车轮不转
    else
        Wheel_Speed = abs(u_ac) / R_eff;
    end
else
    Wheel_Speed = 0; % 空中悬空状态，轮速为 0
end

end
